simulink model "AXU5EV_ADC_HDL"  (R2026b)
settings: Solver=FixedStepDiscrete  StopTime=4e-4  FixedStep=2e-8
libraries: AXU5EV_PL_Algorithm_Library x1
settings Model: Creator=lww  LastModifiedBy=lww

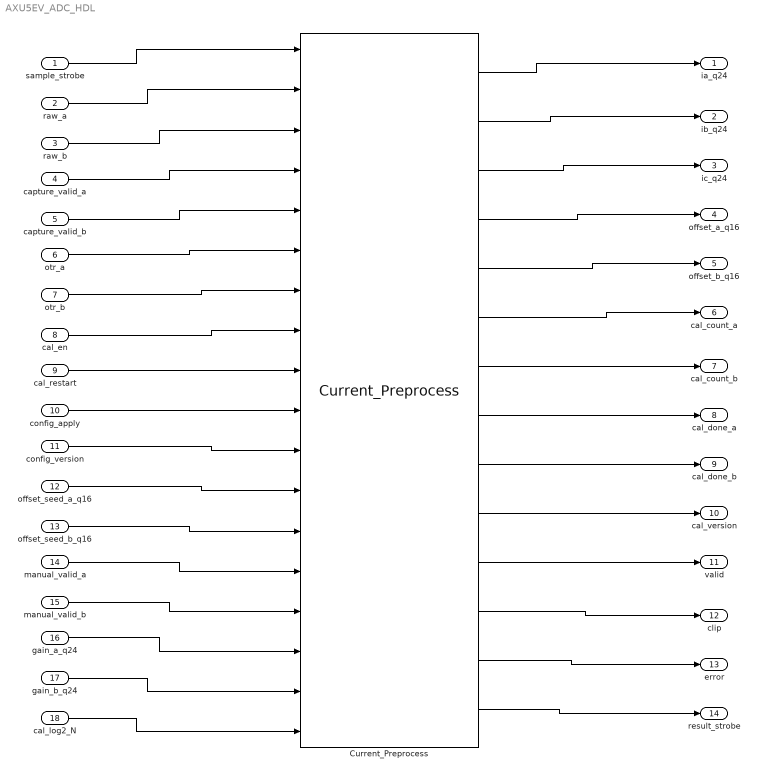
== system AXU5EV_ADC_HDL ==
  sample_strobe : Inport  OutDataTypeStr=boolean  SampleTime=2e-8
  raw_a : Inport  Port=2  OutDataTypeStr=uint16  SampleTime=2e-8
  raw_b : Inport  Port=3  OutDataTypeStr=uint16  SampleTime=2e-8
  capture_valid_a : Inport  Port=4  OutDataTypeStr=boolean  SampleTime=2e-8
  capture_valid_b : Inport  Port=5  OutDataTypeStr=boolean  SampleTime=2e-8
  otr_a : Inport  Port=6  OutDataTypeStr=boolean  SampleTime=2e-8
  otr_b : Inport  Port=7  OutDataTypeStr=boolean  SampleTime=2e-8
  cal_en : Inport  Port=8  OutDataTypeStr=boolean  SampleTime=2e-8
  cal_restart : Inport  Port=9  OutDataTypeStr=boolean  SampleTime=2e-8
  config_apply : Inport  Port=10  OutDataTypeStr=boolean  SampleTime=2e-8
  config_version : Inport  Port=11  OutDataTypeStr=uint32  SampleTime=2e-8
  offset_seed_a_q16 : Inport  Port=12  OutDataTypeStr=int32  SampleTime=2e-8
  offset_seed_b_q16 : Inport  Port=13  OutDataTypeStr=int32  SampleTime=2e-8
  manual_valid_a : Inport  Port=14  OutDataTypeStr=boolean  SampleTime=2e-8
  manual_valid_b : Inport  Port=15  OutDataTypeStr=boolean  SampleTime=2e-8
  gain_a_q24 : Inport  Port=16  OutDataTypeStr=int32  SampleTime=2e-8
  gain_b_q24 : Inport  Port=17  OutDataTypeStr=int32  SampleTime=2e-8
  cal_log2_N : Inport  Port=18  OutDataTypeStr=uint8  SampleTime=2e-8
  Current_Preprocess : AXU5EV_PL_Algorithm_Library/Current_Preprocess  SystemSampleTime=-1  VariantActivationTime=update diagram  EmptyChoice=off  PassThrough=off  PassThroughVariantControl=(default)  EmptyChoiceVariantControl=(default)  AllowFlexibleInterface=on  Latency=0  AutoFrameSizeCalculation=off
  ia_q24 : Outport
  ib_q24 : Outport  Port=2
  ic_q24 : Outport  Port=3
  offset_a_q16 : Outport  Port=4
  offset_b_q16 : Outport  Port=5
  cal_count_a : Outport  Port=6
  cal_count_b : Outport  Port=7
  cal_done_a : Outport  Port=8
  cal_done_b : Outport  Port=9
  cal_version : Outport  Port=10
  valid : Outport  Port=11
  clip : Outport  Port=12
  error : Outport  Port=13
  result_strobe : Outport  Port=14
  wires:
  Current_Preprocess/14 -> result_strobe/1
  Current_Preprocess/13 -> error/1
  Current_Preprocess/12 -> clip/1
  Current_Preprocess/11 -> valid/1
  Current_Preprocess/10 -> cal_version/1
  Current_Preprocess/9 -> cal_done_b/1
  Current_Preprocess/8 -> cal_done_a/1
  Current_Preprocess/7 -> cal_count_b/1
  Current_Preprocess/6 -> cal_count_a/1
  Current_Preprocess/5 -> offset_b_q16/1
  Current_Preprocess/4 -> offset_a_q16/1
  Current_Preprocess/3 -> ic_q24/1
  Current_Preprocess/2 -> ib_q24/1
  Current_Preprocess/1 -> ia_q24/1
  cal_log2_N/1 -> Current_Preprocess/18
  gain_b_q24/1 -> Current_Preprocess/17
  gain_a_q24/1 -> Current_Preprocess/16
  manual_valid_b/1 -> Current_Preprocess/15
  manual_valid_a/1 -> Current_Preprocess/14
  offset_seed_b_q16/1 -> Current_Preprocess/13
  offset_seed_a_q16/1 -> Current_Preprocess/12
  config_version/1 -> Current_Preprocess/11
  config_apply/1 -> Current_Preprocess/10
  cal_restart/1 -> Current_Preprocess/9
  cal_en/1 -> Current_Preprocess/8
  otr_b/1 -> Current_Preprocess/7
  otr_a/1 -> Current_Preprocess/6
  capture_valid_b/1 -> Current_Preprocess/5
  capture_valid_a/1 -> Current_Preprocess/4
  raw_b/1 -> Current_Preprocess/3
  raw_a/1 -> Current_Preprocess/2
  sample_strobe/1 -> Current_Preprocess/1
